simulink model "EV_ML_THD_SPWM"  (R2024b)
settings: Solver=ode4  StartTime=0.0  StopTime=0.2  FixedStep=1e-06  RelTol=1e-3
libraries: simulink x1
settings Model: Creator=ELCOT  LastModifiedBy=ELCOT

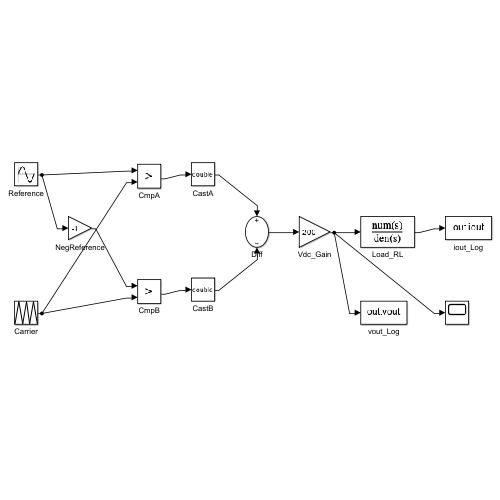
[thumbnail: Simulink's stored preview of the top-level diagram]
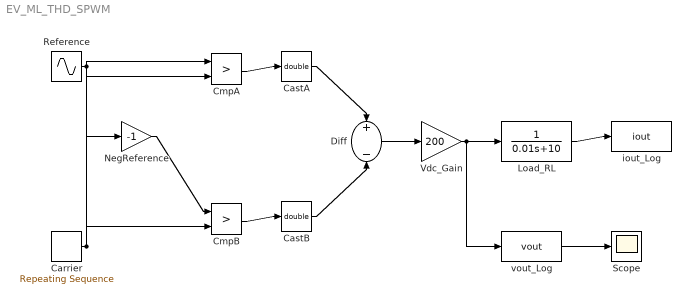
== system EV_ML_THD_SPWM ==
  Carrier : simulink/Sources/Repeating Sequence  rep_seq_t=[0 0.5 1]/9950  rep_seq_y=[-1 1 -1]
  CastA : DataTypeConversion  OutDataTypeStr=double  SaturateOnIntegerOverflow=off  RndMeth=Floor
  CastB : DataTypeConversion  OutDataTypeStr=double  SaturateOnIntegerOverflow=off  RndMeth=Floor
  CmpA : RelationalOperator  Operator=>  OutDataTypeStr=boolean  RndMeth=Simplest  InputSameDT=off
  CmpB : RelationalOperator  Operator=>  OutDataTypeStr=boolean  RndMeth=Simplest  InputSameDT=off
  Diff : Sum  Inputs=+-
  Load_RL : TransferFcn  Numerator=1  Denominator=[0.01 10]
  NegReference : Gain  Gain=-1
  Reference : Sin  Amplitude=0.8  Frequency=314.1593  SampleTime=0
  Scope : Scope
  Vdc_Gain : Gain  Gain=200
  iout_Log : ToWorkspace  VariableName=iout  SaveFormat=Structure With Time  SampleTime=-1
  vout_Log : ToWorkspace  VariableName=vout  SaveFormat=Structure With Time  SampleTime=-1
  wires:
  Reference/1 -> CmpA/1, NegReference/1
  NegReference/1 -> CmpB/1
  Carrier/1 -> CmpA/2, CmpB/2
  CmpA/1 -> CastA/1
  CmpB/1 -> CastB/1
  CastA/1 -> Diff/1
  CastB/1 -> Diff/2
  Diff/1 -> Vdc_Gain/1
  Vdc_Gain/1 -> Load_RL/1, vout_Log/1, Scope/1
  Load_RL/1 -> iout_Log/1
